simulink model "s_b4a4x32kf_26"  (R2018a)
settings: Solver=VariableStepDiscrete  StartTime=0.0  StopTime=10000  RelTol=1e-3
undefined symbols (not defined in the file): fft_stages, n_bits_ants, n_bits_xengs
libraries: xbsIndex_r4 x21247, casper_library_misc x37, casper_library_scopes x13, casper_library_delays x8, xbsReplacements_r4 x6, xps_library x4
(part 41 of 268)

== system s_b4a4x32kf_26/sys2/pipeline8 ==
  d : Inport
  Register0 : xbsIndex_r4/Register  init=0  rst=off  en=off  dbl_ovrd=off  block_type=register
      settings: SourceProductName=The database /home/jmanley/.matlab/R2018a/slblocks_master.db is locked, or a table in the database is locked. (database is locked)  block_version=11.4
  Register1 : xbsIndex_r4/Register  init=0  rst=off  en=off  dbl_ovrd=off  block_type=register
      settings: SourceProductName=The database /home/jmanley/.matlab/R2018a/slblocks_master.db is locked, or a table in the database is locked. (database is locked)  block_version=11.4
  q : Outport
  wires:
  Register0/1 -> Register1/1
  d/1 -> Register0/1
  Register1/1 -> q/1

== system s_b4a4x32kf_26/sys2/pipeline9 ==
  d : Inport
  Register0 : xbsIndex_r4/Register  init=0  rst=off  en=off  dbl_ovrd=off  block_type=register
      settings: SourceProductName=The database /home/jmanley/.matlab/R2018a/slblocks_master.db is locked, or a table in the database is locked. (database is locked)  block_version=11.4
  Register1 : xbsIndex_r4/Register  init=0  rst=off  en=off  dbl_ovrd=off  block_type=register
      settings: SourceProductName=The database /home/jmanley/.matlab/R2018a/slblocks_master.db is locked, or a table in the database is locked. (database is locked)  block_version=11.4
  q : Outport
  wires:
  Register0/1 -> Register1/1
  d/1 -> Register0/1
  Register1/1 -> q/1

== system s_b4a4x32kf_26/sys2/pkt_reord ==
  note: While reading a window out,
      | we erase the contents of that window,
      | and set the MSb (comms error).
  note: BRAM depth is
      | X int length * # antennas * # windows
  din : Inport
  valid_in : Inport  Port=2
  pkt_idx : Inport  Port=3
  time : Inport  Port=4
  ant : Inport  Port=5
  freq : Inport  Port=6
  xeng_id : Inport  Port=7
  Concat : xbsIndex_r4/Concat  num_inputs=2  dbl_ovrd=off  block_type=concat
      settings: SourceProductName=The database /home/jmanley/.matlab/R2018a/slblocks_master.db is locked, or a table in the database is locked. (database is locked)
  Concat1 : xbsIndex_r4/Concat  num_inputs=2  dbl_ovrd=off  block_type=concat
      settings: SourceProductName=The database /home/jmanley/.matlab/R2018a/slblocks_master.db is locked, or a table in the database is locked. (database is locked)
  Concat2 : xbsIndex_r4/Concat  num_inputs=2  dbl_ovrd=off  block_type=concat
      settings: SourceProductName=The database /home/jmanley/.matlab/R2018a/slblocks_master.db is locked, or a table in the database is locked. (database is locked)
  Constant : xbsIndex_r4/Constant  const=0  gui_display_data_type=Fixed-point  arith_type=Unsigned  n_bits=1  bin_pt=0  preci_type=Single  exp_width=8  frac_width=24  explicit_period=on  period=1  equ=P=C  opselect=C  inp2=PCIN>>17  opr=+  inp1=P  carry=CIN  dbl_ovrd=off  block_type=constant
      settings: SourceProductName=The database /home/jmanley/.matlab/R2018a/slblocks_master.db is locked, or a table in the database is locked. (database is locked)
  Constant1 : xbsIndex_r4/Constant  const=2^ant_bits  gui_display_data_type=Fixed-point  arith_type=Unsigned  n_bits=ant_bits+1  bin_pt=0  preci_type=Single  exp_width=8  frac_width=24  explicit_period=on  period=1  equ=P=C  opselect=C  inp2=PCIN>>17  opr=+  inp1=P  carry=CIN  dbl_ovrd=off  block_type=constant
      settings: SourceProductName=The database /home/jmanley/.matlab/R2018a/slblocks_master.db is locked, or a table in the database is locked. (database is locked)
  Constant2 : xbsIndex_r4/Constant  const=1  gui_display_data_type=Fixed-point  arith_type=Unsigned  n_bits=1  bin_pt=0  preci_type=Single  exp_width=8  frac_width=24  explicit_period=on  period=1  equ=P=C  opselect=C  inp2=PCIN>>17  opr=+  inp1=P  carry=CIN  dbl_ovrd=off  block_type=constant
      settings: SourceProductName=The database /home/jmanley/.matlab/R2018a/slblocks_master.db is locked, or a table in the database is locked. (database is locked)
  Constant3 : xbsIndex_r4/Constant  const=2^(x_int_bits-n_bits_input_words)  gui_display_data_type=Fixed-point  arith_type=Unsigned  n_bits=x_int_bits  bin_pt=0  preci_type=Single  exp_width=8  frac_width=24  explicit_period=on  period=1  equ=P=C  opselect=C  inp2=PCIN>>17  opr=+  inp1=P  carry=CIN  dbl_ovrd=off  block_type=constant
      settings: SourceProductName=The database /home/jmanley/.matlab/R2018a/slblocks_master.db is locked, or a table in the database is locked. (database is locked)
  Constant4 : xbsIndex_r4/Constant  const=0  gui_display_data_type=Fixed-point  arith_type=Unsigned  n_bits=n_bits_data  bin_pt=0  preci_type=Single  exp_width=8  frac_width=24  explicit_period=on  period=1  equ=P=C  opselect=C  inp2=PCIN>>17  opr=+  inp1=P  carry=CIN  dbl_ovrd=off  block_type=constant
      settings: SourceProductName=The database /home/jmanley/.matlab/R2018a/slblocks_master.db is locked, or a table in the database is locked. (database is locked)
  Convert : xbsIndex_r4/Convert  gui_display_data_type=Fixed-point  arith_type=Unsigned  n_bits=6  bin_pt=0  float_type=Single  exp_bits=8  fraction_bits=24  quantization=Truncate  overflow=Wrap  en=off  latency=0  pipeline=off  dbl_ovrd=off  block_type=convert
      settings: SourceProductName=The database /home/jmanley/.matlab/R2018a/slblocks_master.db is locked, or a table in the database is locked. (database is locked)
  Counter1 : xbsIndex_r4/Counter  cnt_type=Free Running  cnt_to=1023  operation=Up  start_count=0  cnt_by_val=1  arith_type=Unsigned  n_bits=6  bin_pt=0  load_pin=off  rst=on  en=on  explicit_period=on  period=1  use_behavioral_HDL=on  implementation=Fabric  use_rpm=on  dbl_ovrd=off  block_type=counter
      settings: SourceProductName=The database /home/jmanley/.matlab/R2018a/slblocks_master.db is locked, or a table in the database is locked. (database is locked)  xl_area=[0, 0, 0, 0, 0, 0, 0]
  Delay1 : xbsIndex_r4/Delay  rst=off  infoeditControl=Selection of Reset will increase slice count due to use of real FFs and instead of SRLs  en=off  latency=3  reg_retiming=on  dbl_ovrd=off  block_type=delay
      settings: SourceProductName=The database /home/jmanley/.matlab/R2018a/slblocks_master.db is locked, or a table in the database is locked. (database is locked)  infoedit=Hardware notes: A delay line is a chain, each link of which is an SRL16 or SRL32 followed by a flip-flop.  xl_area=[0, 0, 0, 0, 0, 0, 0]
  Delay10 : Subsystem  Tag=cmac_delinked  mask(pipeline){csp_latency=3}
      mask prompts: csp_latency "Latency"
      mask help:
      | An explicitly laid-out delay line to avoid mapping to SRL16s
      | for use in pipelining to help achieve timing closure.
      mask init:
      | pipeline_init(gcb,'latency',csp_latency);
      settings: AttributesFormatString=Latency = %<latency>
      mask Display:
      | port_label('input', 1, 'd');
      | port_label('output', 1, 'q');
      | disp(['Z^-', num2str(csp_latency)]);
  Delay11 : Subsystem  Tag=cmac_delinked  mask(pipeline){csp_latency=2}
      mask prompts: csp_latency "Latency"
      mask help:
      | An explicitly laid-out delay line to avoid mapping to SRL16s
      | for use in pipelining to help achieve timing closure.
      mask init:
      | pipeline_init(gcb,'latency',csp_latency);
      settings: AttributesFormatString=Latency = %<latency>
      mask Display:
      | port_label('input', 1, 'd');
      | port_label('output', 1, 'q');
      | disp(['Z^-', num2str(csp_latency)]);
  Delay12 : Subsystem  Tag=cmac_delinked  mask(pipeline){csp_latency=2}
      mask prompts: csp_latency "Latency"
      mask help:
      | An explicitly laid-out delay line to avoid mapping to SRL16s
      | for use in pipelining to help achieve timing closure.
      mask init:
      | pipeline_init(gcb,'latency',csp_latency);
      settings: AttributesFormatString=Latency = %<latency>
      mask Display:
      | port_label('input', 1, 'd');
      | port_label('output', 1, 'q');
      | disp(['Z^-', num2str(csp_latency)]);
  Delay13 : Subsystem  Tag=cmac_delinked  mask(pipeline){csp_latency=2}
      mask prompts: csp_latency "Latency"
      mask help:
      | An explicitly laid-out delay line to avoid mapping to SRL16s
      | for use in pipelining to help achieve timing closure.
      mask init:
      | pipeline_init(gcb,'latency',csp_latency);
      settings: AttributesFormatString=Latency = %<latency>
      mask Display:
      | port_label('input', 1, 'd');
      | port_label('output', 1, 'q');
      | disp(['Z^-', num2str(csp_latency)]);
  Delay15 : Subsystem  Tag=cmac_delinked  mask(pipeline){csp_latency=2}
      mask prompts: csp_latency "Latency"
      mask help:
      | An explicitly laid-out delay line to avoid mapping to SRL16s
      | for use in pipelining to help achieve timing closure.
      mask init:
      | pipeline_init(gcb,'latency',csp_latency);
      settings: AttributesFormatString=Latency = %<latency>
      mask Display:
      | port_label('input', 1, 'd');
      | port_label('output', 1, 'q');
      | disp(['Z^-', num2str(csp_latency)]);
  Delay2 : Subsystem  Tag=cmac_delinked  mask(pipeline){csp_latency=2}
      mask prompts: csp_latency "Latency"
      mask help:
      | An explicitly laid-out delay line to avoid mapping to SRL16s
      | for use in pipelining to help achieve timing closure.
      mask init:
      | pipeline_init(gcb,'latency',csp_latency);
      settings: AttributesFormatString=Latency = %<latency>
      mask Display:
      | port_label('input', 1, 'd');
      | port_label('output', 1, 'q');
      | disp(['Z^-', num2str(csp_latency)]);
  Delay20 : xbsIndex_r4/Delay  rst=off  infoeditControl=Selection of Reset will increase slice count due to use of real FFs and instead of SRLs  en=off  latency=3  reg_retiming=on  dbl_ovrd=off  block_type=delay
      settings: SourceProductName=The database /home/jmanley/.matlab/R2018a/slblocks_master.db is locked, or a table in the database is locked. (database is locked)  infoedit=Hardware notes: A delay line is a chain, each link of which is an SRL16 or SRL32 followed by a flip-flop.  xl_area=[0, 0, 0, 0, 0, 0, 0]
  Delay21 : xbsIndex_r4/Delay  rst=off  infoeditControl=Selection of Reset will increase slice count due to use of real FFs and instead of SRLs  en=off  latency=3  reg_retiming=on  dbl_ovrd=off  block_type=delay
      settings: SourceProductName=The database /home/jmanley/.matlab/R2018a/slblocks_master.db is locked, or a table in the database is locked. (database is locked)  infoedit=Hardware notes: A delay line is a chain, each link of which is an SRL16 or SRL32 followed by a flip-flop.  xl_area=[0, 0, 0, 0, 0, 0, 0]
  Delay23 : xbsIndex_r4/Delay  rst=off  infoeditControl=Selection of Reset will increase slice count due to use of real FFs and instead of SRLs  en=off  latency=2  reg_retiming=on  dbl_ovrd=off  block_type=delay
      settings: SourceProductName=The database /home/jmanley/.matlab/R2018a/slblocks_master.db is locked, or a table in the database is locked. (database is locked)  xl_area=[0, 0, 0, 0, 0, 0, 0]
  Delay24 : xbsIndex_r4/Delay  rst=off  infoeditControl=Selection of Reset will increase slice count due to use of real FFs and instead of SRLs  en=off  latency=2  reg_retiming=on  dbl_ovrd=off  block_type=delay
      settings: SourceProductName=The database /home/jmanley/.matlab/R2018a/slblocks_master.db is locked, or a table in the database is locked. (database is locked)  xl_area=[0, 0, 0, 0, 0, 0, 0]
  Delay25 : xbsIndex_r4/Delay  rst=off  infoeditControl=Selection of Reset will increase slice count due to use of real FFs and instead of SRLs  en=off  latency=2  reg_retiming=on  dbl_ovrd=off  block_type=delay
      settings: SourceProductName=The database /home/jmanley/.matlab/R2018a/slblocks_master.db is locked, or a table in the database is locked. (database is locked)  xl_area=[0, 0, 0, 0, 0, 0, 0]
  Delay6 : Subsystem  Tag=cmac_delinked  mask(pipeline){csp_latency=2}
      mask prompts: csp_latency "Latency"
      mask help:
      | An explicitly laid-out delay line to avoid mapping to SRL16s
      | for use in pipelining to help achieve timing closure.
      mask init:
      | pipeline_init(gcb,'latency',csp_latency);
      settings: AttributesFormatString=Latency = %<latency>
      mask Display:
      | port_label('input', 1, 'd');
      | port_label('output', 1, 'q');
      | disp(['Z^-', num2str(csp_latency)]);
  Delay7 : xbsIndex_r4/Delay  rst=off  infoeditControl=Selection of Reset will increase slice count due to use of real FFs and instead of SRLs  en=off  latency=1  reg_retiming=on  dbl_ovrd=off  block_type=delay
      settings: SourceProductName=The database /home/jmanley/.matlab/R2018a/slblocks_master.db is locked, or a table in the database is locked. (database is locked)  xl_area=[0, 0, 0, 0, 0, 0, 0]
  Delay8 : Subsystem  Tag=cmac_delinked  mask(pipeline){csp_latency=1}
      mask prompts: csp_latency "Latency"
      mask help:
      | An explicitly laid-out delay line to avoid mapping to SRL16s
      | for use in pipelining to help achieve timing closure.
      mask init:
      | pipeline_init(gcb,'latency',csp_latency);
      settings: AttributesFormatString=Latency = %<latency>
      mask Display:
      | port_label('input', 1, 'd');
      | port_label('output', 1, 'q');
      | disp(['Z^-', num2str(csp_latency)]);
  Delay9 : Subsystem  Tag=cmac_delinked  mask(pipeline){csp_latency=2}
      mask prompts: csp_latency "Latency"
      mask help:
      | An explicitly laid-out delay line to avoid mapping to SRL16s
      | for use in pipelining to help achieve timing closure.
      mask init:
      | pipeline_init(gcb,'latency',csp_latency);
      settings: AttributesFormatString=Latency = %<latency>
      mask Display:
      | port_label('input', 1, 'd');
      | port_label('output', 1, 'q');
      | disp(['Z^-', num2str(csp_latency)]);
  Delay97 : Subsystem  Tag=cmac_delinked  mask(pipeline){csp_latency=2}
      mask prompts: csp_latency "Latency"
      mask help:
      | An explicitly laid-out delay line to avoid mapping to SRL16s
      | for use in pipelining to help achieve timing closure.
      mask init:
      | pipeline_init(gcb,'latency',csp_latency);
      settings: AttributesFormatString=Latency = %<latency>
      mask Display:
      | port_label('input', 1, 'd');
      | port_label('output', 1, 'q');
      | disp(['Z^-', num2str(csp_latency)]);
  Inverter : xbsIndex_r4/Inverter  en=off  latency=0  dbl_ovrd=off  block_type=inv
      settings: SourceProductName=The database /home/jmanley/.matlab/R2018a/slblocks_master.db is locked, or a table in the database is locked. (database is locked)
  Logical : xbsIndex_r4/Logical  logical_function=AND  inputs=2  en=off  latency=0  precision=Full  arith_type=Unsigned  n_bits=16  bin_pt=0  align_bp=on  dbl_ovrd=off  block_type=logical
      settings: SourceProductName=The database /home/jmanley/.matlab/R2018a/slblocks_master.db is locked, or a table in the database is locked. (database is locked)
  Logical1 : xbsIndex_r4/Logical  logical_function=AND  inputs=2  en=off  latency=0  precision=Full  arith_type=Unsigned  n_bits=16  bin_pt=0  align_bp=on  dbl_ovrd=off  block_type=logical
      settings: SourceProductName=The database /home/jmanley/.matlab/R2018a/slblocks_master.db is locked, or a table in the database is locked. (database is locked)
  Register : xbsIndex_r4/Register  init=0  rst=on  en=on  dbl_ovrd=off  block_type=register
      settings: SourceProductName=The database /home/jmanley/.matlab/R2018a/slblocks_master.db is locked, or a table in the database is locked. (database is locked)
  Slice : xbsIndex_r4/Slice  nbits=16  boolean_output=off  mode=Two Bit Locations  bit1=0  base1=MSB of Input  bit0=x_int_bits  base0=LSB of Input  dbl_ovrd=off  block_type=slice
      settings: SourceProductName=The database /home/jmanley/.matlab/R2018a/slblocks_master.db is locked, or a table in the database is locked. (database is locked)  block_version=10.1.3
  Subsystem7 : Subsystem  mask{clk_rate=240e6}
      mask prompts: clk_rate "board clock rate (Hz)"
  Terminator1 : Terminator
  ant_check : xbsIndex_r4/Assert  assert_type=on  type_source=Explicitly  gui_display_data_type=Fixed-point  arith_type=Unsigned  n_bits=ant_bits  bin_pt=0  preci_type=Single  exp_width=8  frac_width=24  assert_rate=off  rate_source=Explicitly  period=1  output_port=on  block_type=assert
      settings: SourceProductName=The database /home/jmanley/.matlab/R2018a/slblocks_master.db is locked, or a table in the database is locked. (database is locked)
  ant_cnt : xbsIndex_r4/Counter  cnt_type=Free Running  cnt_to=1023  operation=Up  start_count=0  cnt_by_val=1  arith_type=Unsigned  n_bits=x_int_bits + ant_bits  bin_pt=0  load_pin=off  rst=on  en=on  explicit_period=on  period=1  use_behavioral_HDL=on  implementation=Fabric  use_rpm=on  dbl_ovrd=off  block_type=counter
      settings: SourceProductName=The database /home/jmanley/.matlab/R2018a/slblocks_master.db is locked, or a table in the database is locked. (database is locked)  xl_area=[0, 0, 0, 0, 0, 0, 0]
  bus_expand : Subsystem  mask(bus_expand){mode=divisions of arbitrary size, outputNum=1, outputWidth=[2^n_bits_output_words, (2^n_bits_output_words)*n_bits_data], outputBinaryPt=[0, 0], outputArithmeticType=[2, 0], show_format=off, outputToWorkspace=off, variablePrefix=out, outputToModelAsWell=on}
      mask prompts: outputNum "Number of outputs:"; outputWidth "Output width [msb ... lsb]:"; outputBinaryPt "Output binary point position [msb ... lsb]:"; outputArithmeticType "Output arithmetic type (ufix=0, fix=1, bool=2) [msb ... lsb]:"; show_format "Print format string?"; outputToWorkspace "Output to workspace?"; variablePrefix "Variable name prefix:"; outputToModelAsWell "Output to model as well?"
      mask help:
      | Expands a 'bus' made using a bus_create or Xilinx
      | concat block.
      | The input will be divided into the specified number
      | of outputs with the specified arithmetic types.
      | Divisions are made from most significant bit.
      mask init: same as s_b4a4x32kf_26/bus_expand
      settings: AttributesFormatString=2 outputs
      mask TypeOptions mode: divisions of equal size | divisions of arbitrary size
      mask Callback mode: bus_expand_callback();
      mask Callback outputWidth: bus_expand_callback();
      mask Callback outputToWorkspace: bus_expand_callback();
  bus_replicate : Subsystem  Tag=cmac_delinked  mask(bus_replicate){replication=2^n_bits_output_words, csp_latency=0, misc=off, implementation=behavioral}
      mask prompts: replication "replication factor"; csp_latency "latency"; misc "misc support"; implementation "delay implementation"
      mask help: Output bus formed by replicating input bus a number of times
      mask init:
      | bus_replicate_init(gcb, ...
      |     'replication', replication, ...
      |     'csp_latency', csp_latency, ...
      |     'implementation', implementation, ...
      |     'misc', misc);
      mask TypeOptions implementation: core | behavioral
  data_buffer : xbsIndex_r4/Dual Port RAM  depth=2^x_int_bits * 2^ant_bits * 2^window_bits  initVector=zeros(1, 2^x_int_bits * 2^ant_bits * 2^window_bits)  distributed_mem=Block RAM  init_a=0  init_b=0  rst_a=off  rst_b=off  en_a=off  en_b=off  latency=3  write_mode_A=Read Before Write  write_mode_B=Read Before Write  optimize=Speed  dbl_ovrd=off  block_type=dpram
      settings: SourceProductName=The database /home/jmanley/.matlab/R2018a/slblocks_master.db is locked, or a table in the database is locked. (database is locked)  xl_area=[0, 0, 0, 0, 0, 0, 0]  block_version=10.1.3
  data_check : xbsIndex_r4/Assert  assert_type=on  type_source=Explicitly  gui_display_data_type=Fixed-point  arith_type=Unsigned  n_bits=n_bits_data * 2^n_bits_input_words  bin_pt=0  preci_type=Single  exp_width=8  frac_width=24  assert_rate=off  rate_source=Explicitly  period=1  output_port=on  block_type=assert
      settings: SourceProductName=The database /home/jmanley/.matlab/R2018a/slblocks_master.db is locked, or a table in the database is locked. (database is locked)
  freq_check : xbsIndex_r4/Assert  assert_type=on  type_source=Explicitly  gui_display_data_type=Fixed-point  arith_type=Unsigned  n_bits=chan_bits-xeng_bits  bin_pt=0  preci_type=Single  exp_width=8  frac_width=24  assert_rate=off  rate_source=Explicitly  period=1  output_port=on  block_type=assert
      settings: SourceProductName=The database /home/jmanley/.matlab/R2018a/slblocks_master.db is locked, or a table in the database is locked. (database is locked)
  input_control : Subsystem
  munge : Subsystem  mask(munge){divisions=1 + 2^n_bits_input_words, div_size=[1, repmat(n_bits_data, 1, 2^n_bits_input_words)], order=reshape([zeros(1, 2^n_bits_input_words); (1+2^n_bits_input_words)-(1:2^n_bits_input_words)], 1, 2^(n_bits_input_words+1)), arith_type_out=Unsigned, bin_pt_out=0}
      mask prompts: divisions "Number of divisions"; div_size "Division size (bits)"; order "Division packing order"; arith_type_out "Output arithmetic type"; bin_pt_out "Output binary point"
      mask help: Splits an input bus into the specified number of divisions and then recombines them in the order specified (most significant division = 0,least = number divisions-1)
      mask init:
      | munge_init(gcb, ...
      |     'divisions', divisions, ...
      |     'div_size', div_size, ...
      |     'order', order, ...
      |     'arith_type_out', arith_type_out, ...
      |     'bin_pt_out', bin_pt_out);
      settings: AttributesFormatString=|
      | split:[1 32 32 32 32 32 32 32 32]
      | join:[0 8 0 7 0 6 0 5 0 4 0 3 0 2 0 1]
      | Unsigned [264,0]
      mask TypeOptions arith_type_out: Unsigned | Signed  (2's comp) | Floating-point
  munge1 : Subsystem  mask(munge){divisions=2^(n_bits_output_words+1), div_size=reshape([ones(1, 2^n_bits_output_words); repmat(n_bits_data, 1 ,2^n_bits_output_words)], 1, 2^(n_bits_output_words+1)), order=[[0:2:2^(n_bits_output_words+1)-2], [1:2:2^(n_bits_output_words+1)-1]], arith_type_out=Unsigned, bin_pt_out=0}
      mask prompts: divisions "Number of divisions"; div_size "Division size (bits)"; order "Division packing order"; arith_type_out "Output arithmetic type"; bin_pt_out "Output binary point"
      mask help: Splits an input bus into the specified number of divisions and then recombines them in the order specified (most significant division = 0,least = number divisions-1)
      mask init:
      | munge_init(gcb, ...
      |     'divisions', divisions, ...
      |     'div_size', div_size, ...
      |     'order', order, ...
      |     'arith_type_out', arith_type_out, ...
      |     'bin_pt_out', bin_pt_out);
      settings: AttributesFormatString=|
      | split:[1 32]
      | join:[0 1]
      | Unsigned [33,0]
      mask TypeOptions arith_type_out: Unsigned | Signed  (2's comp) | Floating-point
  output_control : Subsystem
  status0 : Subsystem  Tag=xps:sw_reg  AncestorBlock=xps_library/Memory/software_register  mask(swreg){io_dir=To Processor, io_delay=1, init_val=0, sample_period=1, names=[sync_cnt last_missed_ant missed_err_cnt timeout_err_cnt discard_err_cnt], bitwidths=6, bin_pts=0, arith_types=0, sim_port=off, show_format=off}
      mask prompts: io_dir "I/O direction"; io_delay "I/O delay"; init_val "Initial Value"; sample_period "Sample period"; names "Bitfield names [msb...lsb]"; bitwidths "Bitfield widths"; bin_pts "Bitfield binary pts"; arith_types "Bitfield types, ufix=0, fix=1, bool=2"; sim_port "Provide sim input/output?"; show_format "Print format string?"
      mask help: A 32-bit software-accessible register. Can be divided into bitfields of varying widths and types using the fields in the block mask.
      mask init:
      | swreg_init(gcb)
      settings: AttributesFormatString=5 outputs
      mask TypeOptions io_dir: To Processor | From Processor
      mask Callback io_dir:
      | mask_enables = get_param(gcb, 'MaskEnables');
      | mask_names = get_param(gcb, 'MaskNames');
      | if strcmp(get_param(gcb, 'io_dir'), 'To Processor'),
      |     mask_enables{ismember(mask_names, 'sample_period')} = 'off';
      | else
      |     mask_enables{ismember(mask_names, 'sample_period')} = 'on';
      | end
      | set_param(gcb, 'MaskEnables', mask_enables);
      mask DialogControl ParameterTabVar0 Prompt: Setup
  status1 : Subsystem  Tag=xps:sw_reg  AncestorBlock=xps_library/Memory/software_register  mask(swreg){io_dir=To Processor, io_delay=0, init_val=0, sample_period=1, names=dv_per_sec, bitwidths=32, bin_pts=0, arith_types=0, sim_port=off, show_format=on}
      mask prompts: io_dir "I/O direction"; io_delay "I/O delay"; init_val "Initial Value"; sample_period "Sample period"; names "Bitfield names [msb...lsb]"; bitwidths "Bitfield widths"; bin_pts "Bitfield binary pts"; arith_types "Bitfield types, ufix=0, fix=1, bool=2"; sim_port "Provide sim input/output?"; show_format "Print format string?"
      mask help: A 32-bit software-accessible register. Can be divided into bitfields of varying widths and types using the fields in the block mask.
      mask init:
      | swreg_init(gcb)
      settings: AttributesFormatString=1output:uf32.0 = 32 bits
      mask TypeOptions io_dir: To Processor | From Processor
      mask Callback io_dir:
      | mask_enables = get_param(gcb, 'MaskEnables');
      | mask_names = get_param(gcb, 'MaskNames');
      | if strcmp(get_param(gcb, 'io_dir'), 'To Processor'),
      |     mask_enables{ismember(mask_names, 'sample_period')} = 'off';
      | else
      |     mask_enables{ismember(mask_names, 'sample_period')} = 'on';
      | end
      | set_param(gcb, 'MaskEnables', mask_enables);
      mask DialogControl ParameterTabVar0 Prompt: Setup
  sync_ctr1 : xbsIndex_r4/Counter  cnt_type=Free Running  cnt_to=1023  operation=Up  start_count=0  cnt_by_val=1  arith_type=Unsigned  n_bits=6  bin_pt=0  load_pin=off  rst=on  en=on  explicit_period=on  period=1  use_behavioral_HDL=off  implementation=Fabric  use_rpm=on  dbl_ovrd=off  block_type=counter
      settings: SourceProductName=The database /home/jmanley/.matlab/R2018a/slblocks_master.db is locked, or a table in the database is locked. (database is locked)  xl_area=[0, 0, 0, 0, 0, 0, 0]
  sync_ctr5 : xbsIndex_r4/Counter  cnt_type=Free Running  cnt_to=1023  operation=Up  start_count=0  cnt_by_val=1  arith_type=Unsigned  n_bits=6  bin_pt=0  load_pin=off  rst=on  en=on  explicit_period=on  period=1  use_behavioral_HDL=on  implementation=Fabric  use_rpm=on  dbl_ovrd=off  block_type=counter
      settings: SourceProductName=The database /home/jmanley/.matlab/R2018a/slblocks_master.db is locked, or a table in the database is locked. (database is locked)  xl_area=[0, 0, 0, 0, 0, 0, 0]
  sync_ctr6 : xbsIndex_r4/Counter  cnt_type=Free Running  cnt_to=1023  operation=Up  start_count=0  cnt_by_val=1  arith_type=Unsigned  n_bits=6  bin_pt=0  load_pin=off  rst=on  en=on  explicit_period=on  period=1  use_behavioral_HDL=on  implementation=Fabric  use_rpm=on  dbl_ovrd=off  block_type=counter
      settings: SourceProductName=The database /home/jmanley/.matlab/R2018a/slblocks_master.db is locked, or a table in the database is locked. (database is locked)  xl_area=[0, 0, 0, 0, 0, 0, 0]
  time_check : xbsIndex_r4/Assert  assert_type=on  type_source=Explicitly  gui_display_data_type=Fixed-point  arith_type=Unsigned  n_bits=n_bits_timestamp  bin_pt=0  preci_type=Single  exp_width=8  frac_width=24  assert_rate=off  rate_source=Explicitly  period=1  output_port=on  block_type=assert
      settings: SourceProductName=The database /home/jmanley/.matlab/R2018a/slblocks_master.db is locked, or a table in the database is locked. (database is locked)
  time_freq_unpack : Subsystem
  sync_out : Outport
  data_out : Outport  Port=2
  valid_out : Outport  Port=3
  time_out : Outport  Port=4
  freq_out : Outport  Port=5
  recvd : Outport  Port=6
  packet_discarded : Outport  Port=7
  mcnt_timeout : Outport  Port=8
  wires:
  time_freq_unpack/2(freq) -> freq_out/1
  time_freq_unpack/1(time) -> time_out/1
  freq/1 -> freq_check/1
  Constant1/1 -> input_control/7(n_src)
  Constant3/1 -> input_control/6(pkt_size)
  output_control/4(rd_timefreq) -> Delay1/1
  input_control/1(maxcnt) -> output_control/1(maxcnt)
  input_control/3(wr_data) -> Delay23/1
  output_control/1(gen_sync) -> Delay20/1
  data_buffer/1 -> munge1/1(din)
  data_buffer/2 -> Terminator1/1
  output_control/2(rd_en) -> data_buffer/3, Delay21/1
  input_control/2(wr_addr) -> Delay24/1
  input_control/4(we) -> Delay25/1
  xeng_id/1 -> time_freq_unpack/2(xeng_id)
  din/1 -> data_check/1
  ant/1 -> ant_check/1
  Concat2/1 -> input_control/4(time_freq)
  Constant2/1 -> Concat/1
  Concat/1 -> munge/1(din)
  Delay23/1 -> Concat/2
  munge/1(dout) -> data_buffer/5
  Constant4/1 -> Concat1/2
  Constant/1 -> Concat1/1
  bus_replicate/1(out) -> data_buffer/2
  Concat1/1 -> bus_replicate/1(in)
  time/1 -> time_check/1
  bus_expand/2(lsb_out1) -> data_out/1
  time_check/1 -> Concat2/1
  freq_check/1 -> Concat2/2
  bus_expand/1(msb_out2) -> Inverter/1, Logical/2
  data_check/1 -> input_control/1(data_in)
  valid_in/1 -> input_control/2(valid)
  pkt_idx/1 -> input_control/3(pkt_idx)
  ant_check/1 -> input_control/5(src)
  Delay1/1 -> time_freq_unpack/1(din)
  munge1/1(dout) -> bus_expand/1(bus_in)
  Delay25/1 -> data_buffer/6
  output_control/3(rd_addr) -> data_buffer/1
  Delay24/1 -> data_buffer/4
  Delay20/1 -> Counter1/2, ant_cnt/1, sync_out/1
  Counter1/1 -> Delay11/1(d)
  Register/1 -> Delay15/1(d)
  ant_cnt/1 -> Slice/1
  Slice/1 -> Delay6/1(d)
  input_control/6(mcnt_timeout) -> Delay97/1(d), mcnt_timeout/1
  Delay97/1(q) -> sync_ctr6/2
  Delay2/1(q) -> sync_ctr5/1, sync_ctr6/1, sync_ctr1/1, Register/2, Counter1/1
  Delay13/1(q) -> sync_ctr5/2
  input_control/5(discarding) -> packet_discarded/1, Delay13/1(d)
  sync_ctr6/1 -> Delay9/1(d)
  sync_ctr5/1 -> Delay10/1(d)
  sync_ctr1/1 -> Delay8/1(d)
  Delay8/1(q) -> status0/3(out_missed_err_cnt)
  Delay9/1(q) -> status0/4(out_timeout_err_cnt)
  Delay10/1(q) -> status0/5(out_discard_err_cnt)
  Delay12/1(q) -> Register/3, sync_ctr1/2
  Logical/1 -> recvd/1
  [cnt_rst] -> Delay2/1(d)
  Delay11/1(q) -> status0/1(out_sync_cnt)
  Delay15/1(q) -> Convert/1
  Convert/1 -> status0/2(out_last_missed_ant)
  Logical1/1 -> Delay12/1(d)
  Inverter/1 -> Logical1/2
  Delay6/1(q) -> Register/1
  Delay7/1 -> Subsystem7/1(dv)
  Delay21/1 -> valid_out/1, Logical/1, Delay7/1, Logical1/1, ant_cnt/2
  Subsystem7/1(per_sec) -> status1/1(out_dv_per_sec)

== system s_b4a4x32kf_26/sys2/pre_process ==
  data_in : Inport
  valid_in : Inport  Port=2
  eof_in : Inport  Port=3
  spead_time48 : Inport  Port=4
  spead_fengid : Inport  Port=5
  dest_xeng : Inport  Port=6
  this_xeng_id : Inport  Port=7
  freq_in : Inport  Port=8
  Delay{3..5,7,9..10} (6 alike) : xbsIndex_r4/Delay  rst=off  infoeditControl=Selection of Reset will increase slice count due to use of real FFs and instead of SRLs  en=off  latency=1  reg_retiming=on  dbl_ovrd=off  block_type=delay
      settings: SourceProductName=The database /home/jmanley/.matlab/R2018a/slblocks_master.db is locked, or a table in the database is locked. (database is locked)  xl_area=[0, 0, 0, 0, 0, 0, 0]
  Logical3 : xbsIndex_r4/Logical  logical_function=AND  inputs=2  en=off  latency=0  precision=Full  arith_type=Unsigned  n_bits=8  bin_pt=2  align_bp=on  dbl_ovrd=off  block_type=logical
      settings: SourceProductName=The database /home/jmanley/.matlab/R2018a/slblocks_master.db is locked, or a table in the database is locked. (database is locked)  xl_area=[0, 0, 0, 0, 0, 0, 0]
  correct_xengine : xbsIndex_r4/Relational  mode=a=b  op_type=Bool  en=off  latency=1  dbl_ovrd=off  block_type=relational
      settings: SourceProductName=The database /home/jmanley/.matlab/R2018a/slblocks_master.db is locked, or a table in the database is locked. (database is locked)  xl_area=[0, 0, 0, 0, 0, 0, 0]  block_version=10.1.3
  xeng : xbsIndex_r4/Slice  nbits=share_bits  boolean_output=off  mode=Lower Bit Location + Width  bit1=0  base1=MSB of Input  bit0=0  base0=LSB of Input  dbl_ovrd=off  block_type=slice
      settings: SourceProductName=The database /home/jmanley/.matlab/R2018a/slblocks_master.db is locked, or a table in the database is locked. (database is locked)  block_version=10.1.3
  data_out : Outport
  valid : Outport  Port=2
  eof_out : Outport  Port=3
  timestamp : Outport  Port=4
  feng_id : Outport  Port=5
  freq_out : Outport  Port=6
  wires:
  Delay3/1 -> Logical3/1
  this_xeng_id/1 -> xeng/1
  Logical3/1 -> valid/1
  valid_in/1 -> Delay3/1
  xeng/1 -> correct_xengine/2
  eof_in/1 -> Delay7/1
  data_in/1 -> Delay5/1
  Delay5/1 -> data_out/1
  Delay4/1 -> freq_out/1
  Delay7/1 -> eof_out/1
  Delay9/1 -> timestamp/1
  Delay10/1 -> feng_id/1
  freq_in/1 -> Delay4/1
  spead_fengid/1 -> Delay10/1
  correct_xengine/1 -> Logical3/2
  spead_time48/1 -> Delay9/1
  dest_xeng/1 -> correct_xengine/1

== system s_b4a4x32kf_26/sys2/vacc ==
  cnt_rst : Inport
  arm : Inport  Port=2
  start_time : Inport  Port=3
  immediate : Inport  Port=4
  acc_len : Inport  Port=5
  data_in : Inport  Port=6
  we : Inport  Port=7
  timestamp_in : Inport  Port=8
  re : Inport  Port=9
  auto_rst_enable : Inport  Port=10
  Convert : xbsIndex_r4/Convert  gui_display_data_type=Fixed-point  arith_type=Unsigned  n_bits=32  bin_pt=0  float_type=Single  exp_bits=8  fraction_bits=24  quantization=Truncate  overflow=Wrap  en=off  latency=1  pipeline=off  dbl_ovrd=off  block_type=convert
      settings: SourceProductName=The database /home/jmanley/.matlab/R2018a/slblocks_master.db is locked, or a table in the database is locked. (database is locked)
  Logical13 : xbsIndex_r4/Logical  logical_function=AND  inputs=2  en=off  latency=0  precision=Full  arith_type=Unsigned  n_bits=16  bin_pt=0  align_bp=on  dbl_ovrd=off  block_type=logical
      settings: SourceProductName=The database /home/jmanley/.matlab/R2018a/slblocks_master.db is locked, or a table in the database is locked. (database is locked)
  Reinterpret1 : xbsIndex_r4/Reinterpret  force_arith_type=on  arith_type=Unsigned  force_bin_pt=on  bin_pt=0  block_type=reinterpret
      settings: SourceProductName=The database /home/jmanley/.matlab/R2018a/slblocks_master.db is locked, or a table in the database is locked. (database is locked)  block_version=10.1.3
  Subsystem : Subsystem  mask{cnt_bits=4}
      mask DialogControl grp12 Prompt: grp1
  delay1 : xbsIndex_r4/Delay  rst=off  infoeditControl=Selection of Reset will increase slice count due to use of real FFs and instead of SRLs  en=off  latency=2  reg_retiming=on  dbl_ovrd=off  block_type=delay
      settings: SourceProductName=The database /home/jmanley/.matlab/R2018a/slblocks_master.db is locked, or a table in the database is locked. (database is locked)
  delay{2,4,6..8,10..12} (8 alike) : xbsIndex_r4/Delay  rst=off  infoeditControl=Selection of Reset will increase slice count due to use of real FFs and instead of SRLs  en=off  latency=1  reg_retiming=on  dbl_ovrd=off  block_type=delay
      settings: SourceProductName=The database /home/jmanley/.matlab/R2018a/slblocks_master.db is locked, or a table in the database is locked. (database is locked)  infoedit=Hardware notes: A delay line is a chain, each link of which is an SRL16 or SRL32 followed by a flip-flop.
  delay3 : xbsIndex_r4/Delay  rst=off  infoeditControl=Selection of Reset will increase slice count due to use of real FFs and instead of SRLs  en=off  latency=2  reg_retiming=on  dbl_ovrd=off  block_type=delay
      settings: SourceProductName=The database /home/jmanley/.matlab/R2018a/slblocks_master.db is locked, or a table in the database is locked. (database is locked)
  edge_detect4 : Subsystem  mask(edge_detect){edge=Rising, polarity=Active High, x_in=[0 0.08 0.08 0.16 0.16 0.24 0.24 0.32 0.32 0.4], y_in=[-1 -1  1  1  1  1  1  1  1  1], x_out=[0.6 0.68 0.68 0.76 0.76 0.84 0.84 0.92 0.92 1], y_out=[-1 -1  1  1 -1 -1 -1 -1 -1 -1]}
      mask prompts: edge "Edge Type"; polarity "Output Polarity"; x_in "Input X Positions"; y_in "Input Y Positions"; x_out "Output X Positions"; y_out "Output Y Positions"
      mask help: Output is active for one-cycle after each edge of the specified type (i.e. rising, falling or both).
      mask init: same as s_b4a4x32kf_26/edge_detect
      settings: AttributesFormatString=|
      | rising edges
      | active high
      mask Help: Output is active for one-cycle after each edge of the specified type (i.e. rising, falling, or both).  Latency is zero.
      mask TypeOptions edge: Rising | Falling | Both
      mask TypeOptions polarity: Active High | Active Low
      mask Display:
      | plot(x_in_num,0.5+y_in_num*0.2);
      | plot(x_out_num,0.5+y_out_num*0.2);
  hmc_vacc : Subsystem  mask{vector_len=(2^ants_bits)*(2^ants_bits +1) /2 * 8 * 2^(freq_bits-xeng_bits-n_inputs), mezz=1, n_bits=n_bits, n_inputs=n_inputs}
      mask prompts: vector_len "Vector length??(# cycles)"; mezz "Which HMC Mezzanine slot?"; n_bits "Data width (bits)"; n_inputs "Simultaneous inputs (2^?)"
      mask help:
      | A vector accumulator for medium length vectors designed for ROACH's QDR memory.
      |
      | Originally designed for the packetised correlator, this block accepts input data of type Fix_32_0. OOB_data_in provides an extra 4 bits that are accumulated seperately (originally designed to keep track of how many "bad" values in a vector were accumulated).
      |
      | Minimum vector length is 2 * burst_length.
      | Minimum burst length is 10 (recommended default is 2^4=16).
      |
      | The vector length does not need to be a multiple of the burst length.
      mask init:
      | vector_bits = ceil(log2(vector_len));
      | set_param([gcb, '/hmc'], 'mez', mezz);
      | 
      | fmtstr = sprintf('Vector Length: %d', vector_len);
      | set_param(gcb, 'AttributesFormatString', fmtstr);
      settings: AttributesFormatString=Vector Length: 81920
      mask TypeOptions mezz: 0 | 1 | 2 | 3
  hmc_vacc_dummy : Subsystem  mask{vector_len=vector_len, mezz=0, n_bits=n_bits, n_inputs=n_inputs}
      mask prompts: vector_len "Vector length??(# cycles)"; mezz "Which HMC Mezzanine slot?"; n_bits "Data width (bits)"; n_inputs "Simultaneous inputs (2^?)"
      mask help:
      | A vector accumulator for medium length vectors designed for ROACH's QDR memory.
      |
      | Originally designed for the packetised correlator, this block accepts input data of type Fix_32_0. OOB_data_in provides an extra 4 bits that are accumulated seperately (originally designed to keep track of how many "bad" values in a vector were accumulated).
      |
      | Minimum vector length is 2 * burst_length.
      | Minimum burst length is 10 (recommended default is 2^4=16).
      |
      | The vector length does not need to be a multiple of the burst length.
      mask init:
      | fmtstr = sprintf('Vector Length: %d', vector_len);
      | set_param(gcb, 'AttributesFormatString', fmtstr);
      settings: AttributesFormatString=Vector Length: 81920
      mask TypeOptions mezz: 0 | 1 | 2 | 3
  pipeline : Subsystem  Tag=cmac_delinked  mask(pipeline){csp_latency=1}
      mask prompts: csp_latency "Latency"
      mask help:
      | An explicitly laid-out delay line to avoid mapping to SRL16s
      | for use in pipelining to help achieve timing closure.
      mask init:
      | pipeline_init(gcb,'latency',csp_latency);
      settings: AttributesFormatString=Latency = %<latency>
      mask Display:
      | port_label('input', 1, 'd');
      | port_label('output', 1, 'q');
      | disp(['Z^-', num2str(csp_latency)]);
  status : Subsystem  Tag=xps:sw_reg  AncestorBlock=xps_library/Memory/software_register  mask(swreg){io_dir=To Processor, io_delay=1, init_val=0, sample_period=1, names=[acc_cnt err_cnt arm_cnt ld_cnt], bitwidths=[12 12 4 4], bin_pts=0, arith_types=0, sim_port=off, show_format=off}
      mask prompts: io_dir "I/O direction"; io_delay "I/O delay"; init_val "Initial Value"; sample_period "Sample period"; names "Bitfield names [msb...lsb]"; bitwidths "Bitfield widths"; bin_pts "Bitfield binary pts"; arith_types "Bitfield types, ufix=0, fix=1, bool=2"; sim_port "Provide sim input/output?"; show_format "Print format string?"
      mask help: A 32-bit software-accessible register. Can be divided into bitfields of varying widths and types using the fields in the block mask.
      mask init:
      | swreg_init(gcb)
      settings: AttributesFormatString=4 outputs
      mask TypeOptions io_dir: To Processor | From Processor
      mask Callback io_dir:
      | mask_enables = get_param(gcb, 'MaskEnables');
      | mask_names = get_param(gcb, 'MaskNames');
      | if strcmp(get_param(gcb, 'io_dir'), 'To Processor'),
      |     mask_enables{ismember(mask_names, 'sample_period')} = 'off';
      | else
      |     mask_enables{ismember(mask_names, 'sample_period')} = 'on';
      | end
      | set_param(gcb, 'MaskEnables', mask_enables);
      mask DialogControl ParameterTabVar0 Prompt: Setup
  time_latch : xbsIndex_r4/Register  init=0  rst=off  en=on  dbl_ovrd=off  block_type=register
      settings: SourceProductName=The database /home/jmanley/.matlab/R2018a/slblocks_master.db is locked, or a table in the database is locked. (database is locked)
  timestamp : Subsystem  Tag=xps:sw_reg  AncestorBlock=xps_library/Memory/software_register  mask(swreg){io_dir=To Processor, io_delay=0, init_val=0, sample_period=1, names=vacc_timestamp, bitwidths=32, bin_pts=0, arith_types=0, sim_port=off, show_format=on}
      mask prompts: io_dir "I/O direction"; io_delay "I/O delay"; init_val "Initial Value"; sample_period "Sample period"; names "Bitfield names [msb...lsb]"; bitwidths "Bitfield widths"; bin_pts "Bitfield binary pts"; arith_types "Bitfield types, ufix=0, fix=1, bool=2"; sim_port "Provide sim input/output?"; show_format "Print format string?"
      mask help: A 32-bit software-accessible register. Can be divided into bitfields of varying widths and types using the fields in the block mask.
      mask init:
      | swreg_init(gcb)
      settings: AttributesFormatString=1output:uf32.0 = 32 bits
      mask TypeOptions io_dir: To Processor | From Processor
      mask Callback io_dir:
      | mask_enables = get_param(gcb, 'MaskEnables');
      | mask_names = get_param(gcb, 'MaskNames');
      | if strcmp(get_param(gcb, 'io_dir'), 'To Processor'),
      |     mask_enables{ismember(mask_names, 'sample_period')} = 'off';
      | else
      |     mask_enables{ismember(mask_names, 'sample_period')} = 'on';
      | end
      | set_param(gcb, 'MaskEnables', mask_enables);
      mask DialogControl ParameterTabVar0 Prompt: Setup
  vacc_monitor1 : Subsystem
  vacc_time : Subsystem
  data_out : Outport
  valid_out : Outport  Port=2
  rb_done : Outport  Port=3
  timestamp_out : Outport  Port=4
  error_out : Outport  Port=5
  pkt_rdy : Outport  Port=6
  wires:
  start_time/1 -> delay11/1
  hmc_vacc/4(RB_done) -> [rb_done], rb_done/1
  we/1 -> time_latch/2, delay6/1
  data_in/1 -> delay7/1
  acc_len/1 -> delay8/1
  arm/1 -> delay10/1
  Reinterpret1/1 -> delay3/1
  delay7/1 -> Reinterpret1/1
  delay6/1 -> vacc_time/3(valid_in), delay1/1
  timestamp_in/1 -> time_latch/1
  immediate/1 -> delay12/1
  [rb_done] -> vacc_time/4(rb_done)
  time_latch/1 -> vacc_time/1(timestamp_in)
  delay8/1 -> vacc_time/2(acc_len), hmc_vacc/2(n_acum), hmc_vacc_dummy/2(n_acum)
  edge_detect4/1(out) -> vacc_monitor1/2(new_acc)
  [err] -> vacc_monitor1/3(error)
  vacc_monitor1/1(acc_cnt) -> status/1(out_acc_cnt)
  vacc_monitor1/2(error_cnt) -> status/2(out_err_cnt)
  [rb_done] -> edge_detect4/1(in)
  Subsystem/1(arm_count) -> status/3(out_arm_cnt)
  Subsystem/2(ld_count) -> status/4(out_ld_cnt)
  cnt_rst/1 -> delay2/1
  [vacc_armed] -> Subsystem/2(armed)
  delay2/1 -> Subsystem/1(cnt_rst1), vacc_monitor1/1(cnt_rst)
  delay10/1 -> vacc_time/5(arm)
  delay11/1 -> vacc_time/6(load_time)
  delay12/1 -> vacc_time/7(immediate)
  hmc_vacc/1(data_out) -> data_out/1
  hmc_vacc/2(valid) -> valid_out/1
  hmc_vacc/5(pkt_rdy) -> pkt_rdy/1
  delay1/1 -> hmc_vacc_dummy/4(valid_data), hmc_vacc/4(valid_data)
  [vacc_armed] -> hmc_vacc/1(rst), hmc_vacc_dummy/1(rst)
  delay3/1 -> hmc_vacc/3(data_in), hmc_vacc_dummy/3(data_in)
  re/1 -> hmc_vacc/5(ack_RB), hmc_vacc_dummy/5(re)
  Convert/1 -> pipeline/1(d)
  vacc_time/1(timestamp_out) -> timestamp_out/1, Convert/1
  pipeline/1(q) -> timestamp/1(out_vacc_timestamp)
  vacc_time/2(armed) -> [vacc_armed]
  Logical13/1 -> vacc_time/8(ext_err)
  delay4/1 -> Logical13/1
  auto_rst_enable/1 -> delay4/1
  [vacc_err] -> Logical13/2
  vacc_time/4(ts_err) -> [err], error_out/1
  hmc_vacc/3(error) -> [vacc_err]
